simulink model "PV_Wind_BESS_Coordination_R3"  (R2026a)
settings: Solver=FixedStepDiscrete  StopTime=5  FixedStep=1e-3
settings Model: Creator=fakebob2004  LastModifiedBy=fakebob2004

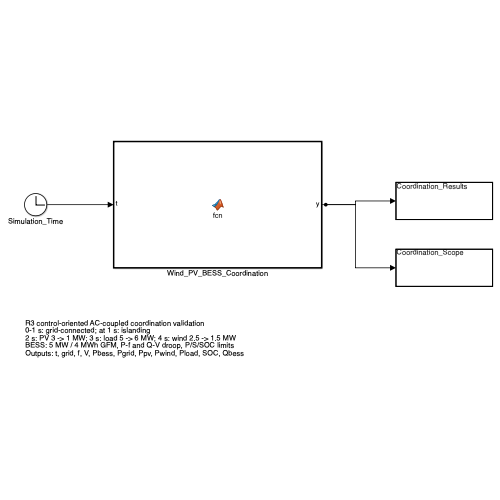
[thumbnail: Simulink's stored preview of the top-level diagram]
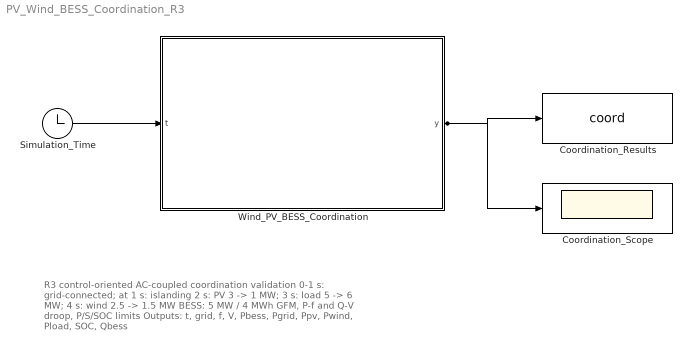
== system PV_Wind_BESS_Coordination_R3 ==
  note: R3 control-oriented AC-coupled coordination validation
      | 0-1 s: grid-connected; at 1 s: islanding
      | 2 s: PV 3 -> 1 MW; 3 s: load 5 -> 6 MW; 4 s: wind 2.5 -> 1.5 MW
      | BESS: 5 MW / 4 MWh GFM, P-f and Q-V droop, P/S/SOC limits
      | Outputs: t, grid, f, V, Pbess, Pgrid, Ppv, Pwind, Pload, SOC, Qbess
  Coordination_Results : ToWorkspace  VariableName=coord  SampleTime=-1
  Coordination_Scope : Scope
  Simulation_Time : Clock
  Wind_PV_BESS_Coordination : MATLAB Function  TreatAsAtomicUnit=on
  wires:
  Simulation_Time/1 -> Wind_PV_BESS_Coordination/1(t)
  Wind_PV_BESS_Coordination/1(y) -> Coordination_Results/1, Coordination_Scope/1

== matlab function PV_Wind_BESS_Coordination_R3/Wind_PV_BESS_Coordination ==
  data: t input; y output
function y = fcn(t)
% Control-oriented wind-PV-BESS island coordination model.
% y = [t grid f_Hz V_pu Pbess_MW Pgrid_MW Ppv_MW Pwind_MW Pload_MW SOC Qbess_Mvar]
%#codegen
persistent fpu vpu pbess_pu soc
Ts = 1e-3; Sbase = 10e6; Ebat_J = 4e6*3600;
H = 2.0; Hq = 0.20; mp = 0.01; nq = 0.10; Tp = 0.05;
Pmax = 0.50; Smax = 0.63; Tgrid = 0.02; Tvgrid = 0.02;
if isempty(fpu)
    fpu = 1.0; vpu = 1.0; pbess_pu = 0.0; soc = 0.60;
end
grid = double(t < 1.0);
if t < 2.0, ppv = 0.30; else, ppv = 0.10; end
if t < 4.0, pwind = 0.25; else, pwind = 0.15; end
if t < 3.0, pload = 0.50; qload = 0.10; else, pload = 0.60; qload = 0.15; end
qpv = ppv*tan(acos(0.90));
pref = min(max((1.0-fpu)/mp, -Pmax), Pmax);
if soc <= 0.20 && pref > 0.0, pref = 0.0; end
if soc >= 0.90 && pref < 0.0, pref = 0.0; end
pbess_pu = pbess_pu + Ts*(pref-pbess_pu)/Tp;
pimb = ppv + pwind + pbess_pu - pload;
if grid > 0.5
    pgrid = -pimb;
    df = (1.0-fpu)/Tgrid;
else
    pgrid = 0.0;
    df = pimb/(2.0*H);
end
fpu = fpu + Ts*df;
qcap = sqrt(max(Smax*Smax-pbess_pu*pbess_pu, 0.0));
qbess = min(max((1.0-vpu)/nq, -qcap), qcap);
qimb = qpv + qbess - qload;
if grid > 0.5
    dv = (1.0-vpu)/Tvgrid;
else
    dv = qimb/(2.0*Hq);
end
vpu = vpu + Ts*dv;
soc = min(max(soc - Ts*pbess_pu*Sbase/Ebat_J, 0.0), 1.0);
y = [t,grid,50.0*fpu,vpu,pbess_pu*Sbase/1e6,pgrid*Sbase/1e6, ...
     ppv*Sbase/1e6,pwind*Sbase/1e6,pload*Sbase/1e6,soc, ...
     qbess*Sbase/1e6];
end
